simulink model "demo_noise"  (R2026a)
settings: Solver=FixedStepDiscrete  StopTime=2  FixedStep=.1
libraries: simulink x1
settings Model: Creator=harry_31916  LastModifiedBy=harry_31916

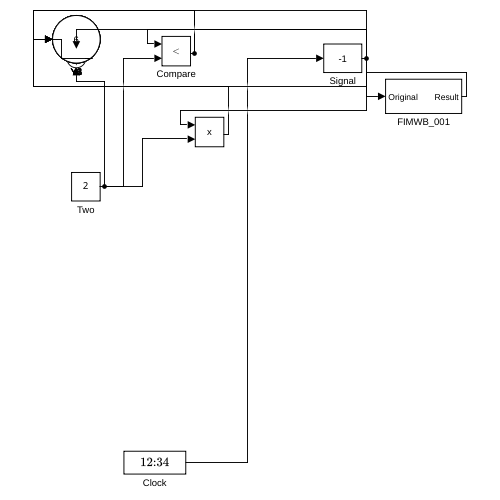
[thumbnail: Simulink's stored preview of the top-level diagram]
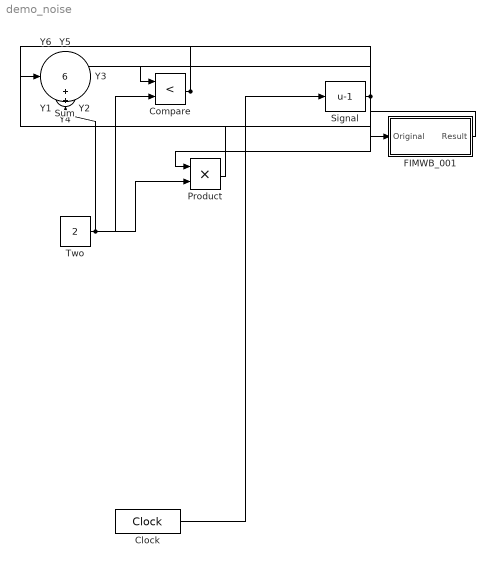
== system demo_noise ==
  Clock : DigitalClock  SampleTime=.1
  Compare : RelationalOperator  Operator=<  OutDataTypeStr=boolean  RndMeth=Simplest  InputSameDT=off
  FIMWB_001 : Subsystem  Tag=fimwb.fault.1
  Product : Product  Inputs=**
  Signal : Bias  Bias=-1  SaturateOnIntegerOverflow=off
  Sum : Sum
  Two : Constant  Value=2
  Y1 : Outport  SampleTime=0.1
  Y2 : Outport  Port=2  SampleTime=0.1
  Y3 : Outport  Port=3  SampleTime=0.1
  Y4 : Outport  Port=4  SampleTime=0.1
  Y5 : Outport  Port=5  SampleTime=0.1
  Y6 : Outport  Port=6  SampleTime=0.1
  wires:
  Clock/1 -> Signal/1
  Signal/1 -> Sum/1, Product/1, Compare/1, Y2/1, FIMWB_001/1(Original)
  Two/1 -> Sum/2, Product/2, Compare/2
  Sum/1 -> Y3/1
  Product/1 -> Y4/1
  Compare/1 -> Y5/1, Y6/1
  FIMWB_001/1(Result) -> Y1/1

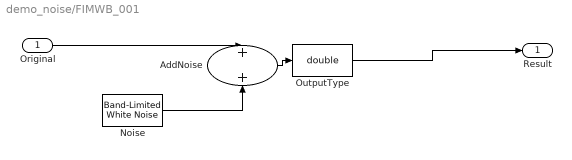
== system demo_noise/FIMWB_001 ==
  Original : Inport
  AddNoise : Sum
  Noise : simulink/Sources/Band-Limited White Noise  Cov=0.01  Ts=0.10000000000000001  seed=1
  OutputType : DataTypeConversion  OutDataTypeStr=double  RndMeth=Round
  Result : Outport
  wires:
  Original/1 -> AddNoise/1
  Noise/1 -> AddNoise/2
  AddNoise/1 -> OutputType/1
  OutputType/1 -> Result/1
